simulink model "DifAndCtrl"  (R2026a)
settings: Solver=FixedStepDiscrete  StopTime=tf  FixedStep=0.01
values from neighbouring files (symbols this model uses):
  ArmConstants = struct('l1_dim', l1_dim,                        'l2_dim', l2_dim,                        'Hexa_to_joint_L', L,                        'Mass1', ml1,                        'Mass2', ml2,                        'Inertia1', Hl1,                        'Inertia2', Hl2,                        'MC1', c1,                        'MC2', c2,                        'Servos', Servos)    [init_model.m]    (also in init_var.m)
  Differentiator = struct('G1', G1 ,     'G2', G2 ,     'Q1', Q1 ,     'Q2', Q2 ,     'w1', w1 ,     'w2', w2 ,     'p1', p1 ,     'p2', p2)    [init_model.m]    (also in init_var.m)
  HexaConstants = struct('Mass', mb,                         'Inertia', J ,                         'allo', allo,                          'invallo', invallo,                         'kT', kT)    [init_model.m]    (also in init_var.m)
undefined symbols (not defined in the file or in its folder): DiscIntNeverNeededParam
settings Model: ExtModeTrigDuration=10  Creator=Carlos Fabian  LastModifiedBy=Carlos Fabian
settings SolverCC: PositivePriorityOrder=on
settings OptimizationCC: UseDivisionForNetSlopeComputation=on  GainParamInheritBuiltInType=on  UseFloatMulNetSlope=on  InlineInvariantSignals=on  NoFixptDivByZeroProtection=on  EfficientFloat2IntCast=on  LifeSpan=1
settings HardwareCC: ProdLargestAtomicInteger=Long  ProdLargestAtomicFloat=Double  ProdHWDeviceType=ARM Compatible->ARM Cortex
settings SFSimCC: SimTargetLang=C++
settings RTWCC: SystemTargetFile=ert.tlc  HardwareBoard=PX4 Pixhawk 6c  TLCOptions="-aInlineSetEventsForThisBaseRateFcn=TLC_FALSE -aSuppressMultiTaskScheduler=TLC_FALSE  -aRateBasedStepFcn=0"  Toolchain=GNU Tools for PX4 Autopilots  TargetLang=C++  Description=Embedded Coder
settings ERTTargetCC: ExtModeTransport=3.0  ExtModeStaticAllocSize=1024.0  RootIOFormat=Structure reference  ERTFilePackagingFormat=CompactWithDataFile  IncludeMdlTerminateFcn=off  CombineSignalStateStructs=on  SuppressErrorStatus=on  CodeInterfacePackaging=C++ class  SubcomponentCodeInterfacePackaging=C++ class  SupportComplex=off
settings ExplorerConfigSet: InternalSimMechanicsExplorerSettings=|
  | <ExplorerConfiguration>
  | 
  |   <canonicalview>default</canonicalview>
  | 
  |   <TilePanel>
  |     <TileInfo>
  |       <Tiles Columns="1" Count="1" Height="513" Rows="1" Width="1199">
  |         <Row Weight="1"/>
  |         <Column Weight="1"/>
  |         <Tile Height="1" Width="1" X="0" Y="0"/>
  |       </Tiles>
  |     </TileInfo>
  |     <SceneInfo>
  |       <SceneViewer>
  |         <IsThisViewStd>
  |           <IsStandardView>off</IsStandardView>
  |           <StandardViewName>Front</StandardViewName>
  |         </IsThisViewStd>
  |         <BGColor>
  |           <R>1</R>
  |           <G>1</G>
  |           <B>1</B>
  |           <A>1</A>
  |         </BGColor>
  |         <Camera>
  |           <DoPerspective>off</DoPerspective>
  |           <Position>
  |             <X>16.563809413425133</X>
  |             <Y>-16.563809413425133</Y>
  |             <Z>17.346953838391503</Z>
  |           </Position>
  |           <Center>
  |             <X>0</X>
  |             <Y>0</Y>
  |             <Z>0.78314442496637693</Z>
  |           </Center>
  |           <Up>
  |             <X>-0.40824829046386285</X>
  |             <Y>0.40824829046386285</Y>
  |             <Z>0.81649658092772603</Z>
  |           </Up>
  |           <XLim>3.39184009237395</XLim>
  |           <YLim>3.39184009237395</YLim>
  |           <ViewLimDist>0.01</ViewLimDist>
  |         </Camera>
  |       </SceneViewer>
  |     </SceneInfo>
  |   </TilePanel>
  | 
  |   <MechEditorPanel>
  |     <GfxPanelCameraMap/>
  |     <Cameras/>
  |     <VideoCreator>
  |       <IncludeTiles>All</IncludeTiles>
  |       <IncludeTime>on</IncludeTime>
  |       <IncludeWorldFrame>off</IncludeWorldFrame>
  |       <PlaybackSpeedRatio>8</PlaybackSpeedRatio>
  |       <FrameRate>24</FrameRate>
  |       <FrameSize>auto</FrameSize>
  |       <VideoFormat>MotionJPEGAVI</VideoFormat>
  |     </VideoCreator>
  |   </MechEditorPanel>
  | 
  |   <PlaybackSettings>
  |     <PlaybackSpeedFactor>4</PlaybackSpeedFactor>
  |   </PlaybackSettings>
  | 
  | </ExplorerConfiguration>

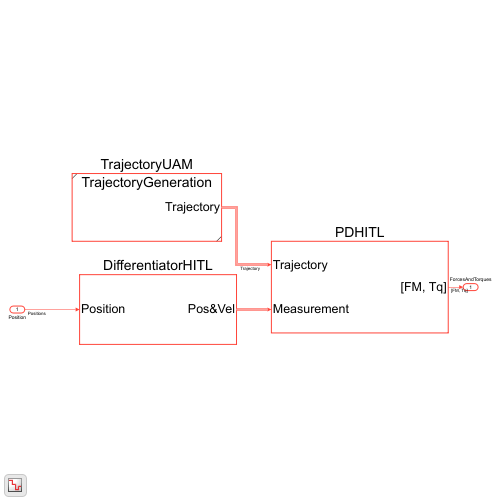
[thumbnail: Simulink's stored preview of the top-level diagram]
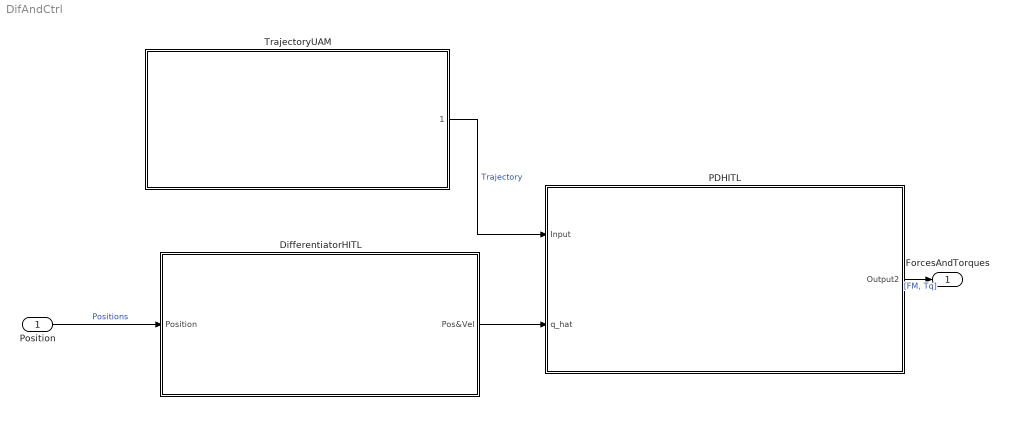
== system DifAndCtrl ==
  Position : Inport  OutDataTypeStr=double  PortDimensions=8  SampleTime=0.01
  DifferentiatorHITL : Subsystem
  PDHITL : Subsystem
  TrajectoryUAM : Subsystem  ReferencedSubsystem=TrajectoryGeneration
  ForcesAndTorques : Outport  OutDataTypeStr=double  PortDimensions=[8 1]  SampleTime=0.01
  wires:
  PDHITL/1(Output2) -> ForcesAndTorques/1  "[FM, Tq]"
  Position/1 -> DifferentiatorHITL/1(Position)  "Positions"
  TrajectoryUAM/1 -> PDHITL/1(Input)  "Trajectory"
  DifferentiatorHITL/1(Pos&Vel) -> PDHITL/2(q_hat)

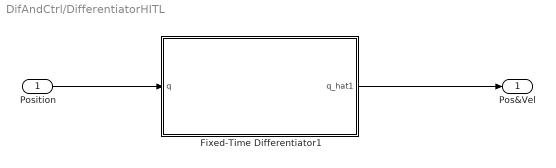
== system DifAndCtrl/DifferentiatorHITL ==
  Position : Inport  SampleTime=0.01
  Fixed-Time Differentiator1 : Subsystem
      settings: PortSchema="{\"entries\":[{\"content\":{\"sides\":[{\"content\":{\"connectorIds\":[\"Out1\"]},\"type\":\"ConnectorPlacement.EquallySpacedRectSide\",\"uuid\":\"d79ec49c-5563-41e0-ac59-6e897bc19fda\"},{\"content\":{\"connectorIds\":[\"In1\"],\"side\":\"RIGHT\"},\"type\":\"ConnectorPlacement.EquallySpacedRectSide\",\"uuid\":\"1255043e-c90e-4bae-9fb4-4fa06f36f53e\"},{\"content\":{\"side\":\"TOP\"},\"type\":\"ConnectorPlacement.EquallySpacedRectSide\",\"uuid\":\"823ada36-3f22-4ee3-87a1-180276f622bc\"}]},\"type\":\"ConnectorPlacement.EquallySpacedConnector\",\"uuid\":\"7403b609-b333-4977-a854-ed7a71f74338\"}],\"packageUris\":[\"http://schema.mathworks.com/mf0/Connector/R2020b\"],\"version\":\"1.0\"}"
  Pos&Vel : Outport
  wires:
  Fixed-Time Differentiator1/1(q_hat1) -> Pos&Vel/1
  Position/1 -> Fixed-Time Differentiator1/1(q)

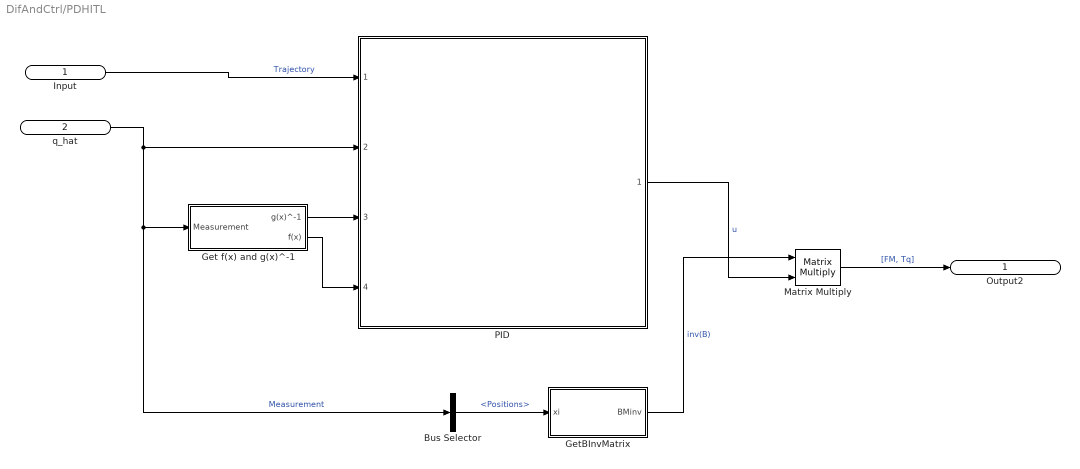
== system DifAndCtrl/PDHITL ==
  Input : Inport
  q_hat : Inport  Port=2
  Bus Selector : BusSelector  OutputSignals=Positions
  Get f(x) and g(x)^-1 : Subsystem
  GetBInvMatrix : MATLAB Function  TreatAsAtomicUnit=on
  Matrix Multiply : Product  Multiplication=Matrix(*)
  PID : Subsystem  ReferencedSubsystem=PIDController
  Output2 : Outport
  wires:
  Get f(x) and g(x)^-1/2(f(x)) -> PID/4
  Get f(x) and g(x)^-1/1(g(x)^-1) -> PID/3
  Matrix Multiply/1 -> Output2/1  "[FM, Tq]"
  PID/1 -> Matrix Multiply/2  "u"
  GetBInvMatrix/1(BMinv) -> Matrix Multiply/1  "inv(B)"
  Bus Selector/1 -> GetBInvMatrix/1(xi)  "<Positions>"
  Input/1 -> PID/1  "Trajectory"
  q_hat/1 -> PID/2, Bus Selector/1, Get f(x) and g(x)^-1/1(Measurement)  "Measurement"

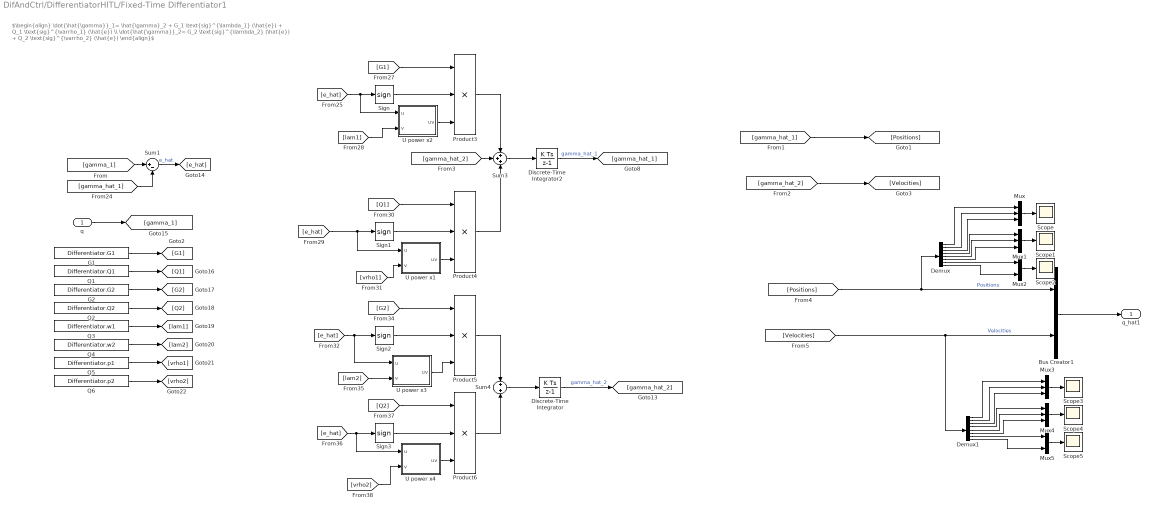
== system DifAndCtrl/DifferentiatorHITL/Fixed-Time Differentiator1 ==
  note: $\begin{align} \dot{\hat{\gamma}}_1= \hat{\gamma}_2 + G_1 \text{sig}^{\lambda_1} (\hat{e}) + Q_1 \text{sig}^{\varrho_1} (\hat{e}) \\ \dot{\hat{\gamma}}_2= G_2 \text{sig}^{\lambda_2} (\hat{e}) + Q_2 \text{sig}^{\varrho_2} (\hat{e}) \end{align}$
  q : Inport  SampleTime=0.01
  Bus Creator1 : BusCreator  Inputs=2
  Demux : Demux  Outputs=8
  Demux1 : Demux  Outputs=8
  Discrete-Time Integrator : DiscreteIntegrator  SampleTime=-1  ICPrevOutput=DiscIntNeverNeededParam  ICPrevScaledInput=DiscIntNeverNeededParam
  Discrete-Time Integrator2 : DiscreteIntegrator  SampleTime=-1  ICPrevOutput=DiscIntNeverNeededParam  ICPrevScaledInput=DiscIntNeverNeededParam
  G1 : Constant  Value=Differentiator.G1
  G2 : Constant  Value=Differentiator.G2
  Mux{,1,3..4} (4 alike) : Mux  Inputs=3
  Mux2 : Mux  Inputs=2
  Mux5 : Mux  Inputs=2
  Product{3..6} (4 alike) : Product  Inputs=3
  Q1 : Constant  Value=Differentiator.Q1
  Q2 : Constant  Value=Differentiator.Q2
  Q3 : Constant  Value=Differentiator.w1
  Q4 : Constant  Value=Differentiator.w2
  Q5 : Constant  Value=Differentiator.p1
  Q6 : Constant  Value=Differentiator.p2
  Scope{,1..5} (6 alike) : Scope
      Scope2 settings: DataLoggingVariableName=ScopeData2
      Scope3 settings: DataLoggingVariableName=ScopeData3
      Scope4 settings: DataLoggingVariableName=ScopeData4
      Scope5 settings: DataLoggingVariableName=ScopeData5
  Sign{,1..3} (4 alike) : Signum
  Sum1 : Sum  Inputs=|+-
  Sum3 : Sum  Inputs=+++
  Sum4 : Sum  Inputs=+|+
  U power x1 : MATLAB Function  TreatAsAtomicUnit=on
  U power x2 : MATLAB Function  TreatAsAtomicUnit=on
  U power x3 : MATLAB Function  TreatAsAtomicUnit=on
  U power x4 : MATLAB Function  TreatAsAtomicUnit=on
  q_hat1 : Outport
  wires:
  Discrete-Time Integrator/1 -> [gamma_hat_2]  "gamma_hat_2"
  [Velocities] -> Demux1/1, Bus Creator1/2  "Velocities"
  [Positions] -> Demux/1, Bus Creator1/1  "Positions"
  Bus Creator1/1 -> q_hat1/1
  [gamma_hat_1] -> [Positions]
  U power x4/1(uv) -> Product6/3
  U power x3/1(uv) -> Product5/3
  U power x1/1(uv) -> Product4/3
  [lam1] -> U power x2/2(v)
  U power x2/1(uv) -> Product3/3
  [e_hat] -> Sign/1, U power x2/1(u)
  [e_hat] -> Sign3/1, U power x4/1(u)
  [e_hat] -> Sign2/1, U power x3/1(u)
  [e_hat] -> Sign1/1, U power x1/1(u)
  [Q1] -> Product4/1
  [vrho1] -> U power x1/2(v)
  Sign1/1 -> Product4/2
  Product4/1 -> Sum3/3
  [gamma_hat_2] -> Sum3/2
  Sum3/1 -> Discrete-Time Integrator2/1
  Sum4/1 -> Discrete-Time Integrator/1
  [gamma_hat_2] -> [Velocities]
  Discrete-Time Integrator2/1 -> [gamma_hat_1]  "gamma_hat_1"
  q/1 -> [gamma_1]
  Q3/1 -> [lam1]
  Sign/1 -> Product3/2
  Product3/1 -> Sum3/1
  [Q2] -> Product6/1
  [G2] -> Product5/1
  [lam2] -> U power x3/2(v)
  [gamma_1] -> Sum1/1
  Product5/1 -> Sum4/1
  Q4/1 -> [lam2]
  Sign2/1 -> Product5/2
  G2/1 -> [G2]
  [G1] -> Product3/1
  Q2/1 -> [Q2]
  [vrho2] -> U power x4/2(v)
  Q6/1 -> [vrho2]
  Q1/1 -> [Q1]
  Q5/1 -> [vrho1]
  [gamma_hat_1] -> Sum1/2
  Sign3/1 -> Product6/2
  Sum1/1 -> [e_hat]  "e_hat"
  G1/1 -> [G1]
  Product6/1 -> Sum4/2
  Mux/1 -> Scope/1
  Mux1/1 -> Scope1/1
  Mux2/1 -> Scope2/1
  Demux/1 -> Mux/1
  Demux/2 -> Mux/2
  Demux/3 -> Mux/3
  Demux/4 -> Mux1/1
  Demux/5 -> Mux1/2
  Demux/6 -> Mux1/3
  Demux/7 -> Mux2/1
  Demux/8 -> Mux2/2
  Demux1/3 -> Mux3/3
  Demux1/2 -> Mux3/2
  Demux1/6 -> Mux4/3
  Demux1/5 -> Mux4/2
  Mux5/1 -> Scope5/1
  Demux1/1 -> Mux3/1
  Demux1/4 -> Mux4/1
  Demux1/8 -> Mux5/2
  Demux1/7 -> Mux5/1
  Mux3/1 -> Scope3/1
  Mux4/1 -> Scope4/1

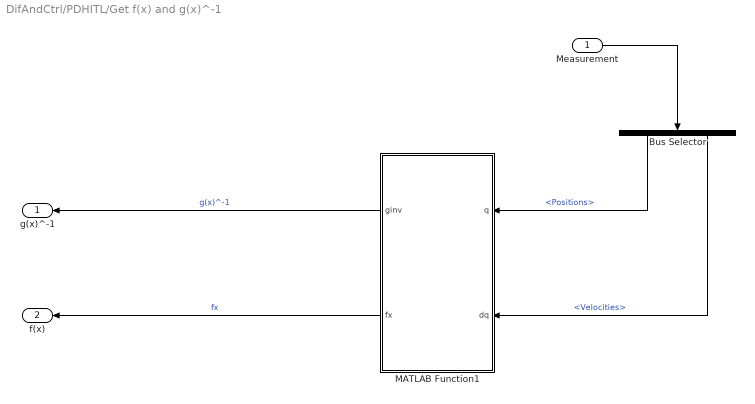
== system DifAndCtrl/PDHITL/Get f(x) and g(x)^-1 ==
  Measurement : Inport
  Bus Selector : BusSelector  OutputSignals=Positions,Velocities
  MATLAB Function1 : MATLAB Function  TreatAsAtomicUnit=on
  g(x)^-1 : Outport
  f(x) : Outport  Port=2
  wires:
  Bus Selector/2 -> MATLAB Function1/2(dq)  "<Velocities>"
  Bus Selector/1 -> MATLAB Function1/1(q)  "<Positions>"
  Measurement/1 -> Bus Selector/1
  MATLAB Function1/1(ginv) -> g(x)^-1/1  "g(x)^-1"
  MATLAB Function1/2(fx) -> f(x)/1  "fx"

== matlab function DifAndCtrl/PDHITL/GetBInvMatrix ==
  data: xi input; BMinv output
function BMinv = GetBInvMatrix(xi)

% phi = xi(4);
% th  = xi(5);
% psi = xi(6);
% 
% BM1=[cos(phi)*cos(th),-cos(phi)*sin(psi)+cos(psi)*sin(phi)*sin(th), ...
%     sin(phi)*sin(psi)+cos(phi)*cos(psi)*sin(th),0,0,0;...
%     cos(th)*sin(psi), cos(phi)*cos(psi)+sin(phi)*sin(psi)*sin(th),...
%     -cos(psi)*sin(phi)+cos(phi)*sin(psi)*sin(phi),0,0,0;...
%     -sin(th),cos(th)*sin(psi),cos(phi)*cos(th),0,0,0;...
%     0,0,0,1,sin(phi)*tan(th),cos(phi)*tan(th);...
%     0,0,0,0,cos(phi),-sin(phi);0,0,0,0,sec(th)*sin(phi),cos(phi)*sec(th)];

BM1 = BMatrix(xi);

BM = blkdiag(BM1, eye(2,2));

BMinv = inv(BM);

end

== matlab function DifAndCtrl/DifferentiatorHITL/Fixed-Time Differentiator1/U power x2 ==
  data: u input; uv output; v input
function uv = u_x(u, v)
i = 1;
uv = zeros(8,1);
for i=1:8
    absolute = abs(u(i));
    uv(i) = absolute ^ v(i);
    % if absolute < 0.00005
    %     uv(i) = 0;
    % else
    %     uv(i) = absolute ^ v(i);
    % end
end
end

== matlab function DifAndCtrl/DifferentiatorHITL/Fixed-Time Differentiator1/U power x1 ==
  data: u input; uv output; v input
function uv = u_x(u, v)
i = 1;
uv = zeros(8,1);
for i=1:8
    absolute = abs(u(i));
    uv(i) = absolute ^ v(i);
    % if absolute < 0.00005
    %     uv(i) = 0;
    % else
    %     uv(i) = absolute ^ v(i);
    % end
end
end

== matlab function DifAndCtrl/DifferentiatorHITL/Fixed-Time Differentiator1/U power x3 ==
  data: u input; uv output; v input
function uv = u_x(u, v)
i = 1;
uv = zeros(8,1);
for i=1:8
    absolute = abs(u(i));
    uv(i) = absolute ^ v(i);
    % if absolute < 0.00005
    %     uv(i) = 0;
    % else
    %     uv(i) = absolute ^ v(i);
    % end
end
end

== matlab function DifAndCtrl/DifferentiatorHITL/Fixed-Time Differentiator1/U power x4 ==
  data: u input; uv output; v input
function uv = u_x(u, v)
i = 1;
uv = zeros(8,1);
for i=1:8
    absolute = abs(u(i));
    uv(i) = absolute ^ v(i);
    % if absolute < 0.00005
    %     uv(i) = 0;
    % else
    %     uv(i) = absolute ^ v(i);
    % end
end
end

== matlab function DifAndCtrl/PDHITL/Get f(x) and g(x)^-1/MATLAB Function1 ==
  data: q input; dq input; HexaConstants parameter; ginv output; fx output; ArmConstants parameter
function [ginv, fx] = Get_DCG_Hexa(q, dq, HexaConstants, ArmConstants)

DM = DMatrix(q, HexaConstants, ArmConstants);
CM = CMatrix(q, dq, HexaConstants, ArmConstants);
Gv = GVector(q, HexaConstants, ArmConstants);

ginv = DM;

fx = DM\( -CM*dq - Gv );

end
